simulink model "DataCenterHeatReuse_Core"  (R2026a)
settings: Solver=FixedStepDiscrete  StopTime=24  FixedStep=1
settings Model: Creator=Lysda  LastModifiedBy=Lysda

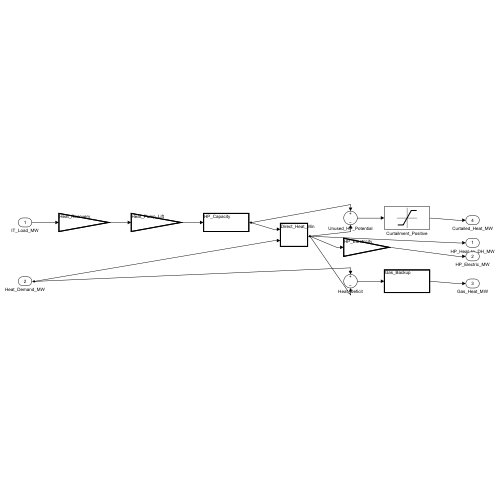
[thumbnail: Simulink's stored preview of the top-level diagram]
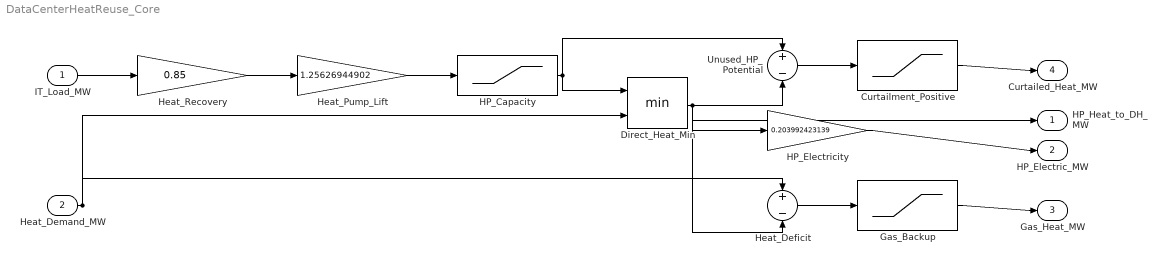
== system DataCenterHeatReuse_Core ==
  IT_Load_MW : Inport
  Heat_Demand_MW : Inport  Port=2
  Curtailment_Positive : Saturate  UpperLimit=inf  LowerLimit=0
  Direct_Heat_Min : MinMax  Inputs=2
  Gas_Backup : Saturate  UpperLimit=inf  LowerLimit=0
  HP_Capacity : Saturate  UpperLimit=12  LowerLimit=0
  HP_Electricity : Gain  Gain=0.203992423139
  Heat_Deficit : Sum  Inputs=+-
  Heat_Pump_Lift : Gain  Gain=1.25626944902
  Heat_Recovery : Gain  Gain=0.85
  Unused_HP_Potential : Sum  Inputs=+-
  HP_Heat_to_DH_MW : Outport
  HP_Electric_MW : Outport  Port=2
  Gas_Heat_MW : Outport  Port=3
  Curtailed_Heat_MW : Outport  Port=4
  wires:
  IT_Load_MW/1 -> Heat_Recovery/1
  Heat_Recovery/1 -> Heat_Pump_Lift/1
  Heat_Pump_Lift/1 -> HP_Capacity/1
  HP_Capacity/1 -> Direct_Heat_Min/1, Unused_HP_Potential/1
  Heat_Demand_MW/1 -> Direct_Heat_Min/2, Heat_Deficit/1
  Direct_Heat_Min/1 -> Heat_Deficit/2, Unused_HP_Potential/2, HP_Electricity/1, HP_Heat_to_DH_MW/1
  Heat_Deficit/1 -> Gas_Backup/1
  Unused_HP_Potential/1 -> Curtailment_Positive/1
  HP_Electricity/1 -> HP_Electric_MW/1
  Gas_Backup/1 -> Gas_Heat_MW/1
  Curtailment_Positive/1 -> Curtailed_Heat_MW/1
